simulink model "AFC_FFNN_trainscg_15_15_15_15_15_ctr_Nor_July_15"  (R2021a)
settings: Solver=VariableStepAuto  StartTime=0.0  StopTime=10.0  RelTol=1e-3
libraries: neural x82
(part 1 of 3)
settings Model: Creator=deyun  LastModifiedBy=deyun

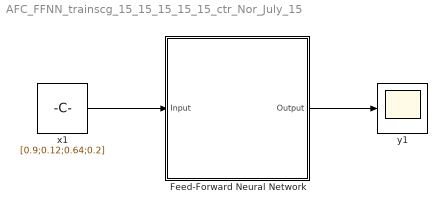
== system AFC_FFNN_trainscg_15_15_15_15_15_ctr_Nor_July_15 ==
  Feed-Forward Neural Network : Subsystem
      mask help: Feed-Forward Neural Network
      mask Display: e = 0.06;c1 = [120 150 230]/255;c2 = ([120 150 230]+0)/383;c3 = ([120 150 230]+128)/383;patch([0 1 1 0],[0 0 1 1],c1);patch([0 1 1 1-e 1-e 0+e],[0 0 1 1-e 0+e 0+e],c2);patch([0 0 1 1-e 0+e 0+e],[0 1 1 1-e 1-e 0+e],c3);plot([0 1 1 0 0],[0 0 1 1 0]);fprintf('NNET');port_label('input',1,' Input');port_label('output',1,'Output ');
  x1 : Constant  Value=[0.9;0.12;0.64;0.2]  SampleTime=1
      mask Display: e = 0.06;c1 = [120 230 180]/255;c2 = ([120 230 180]+0)/(256+128);c3 = ([120 230 180]+128)/(256+128);patch([0 1 1 0],[0 0 1 1],c1);patch([0 1 1 1-e 1-e 0+e],[0 0 1 1-e 0+e 0+e],c2);patch([0 0 1 1-e 0+e 0+e],[0 1 1 1-e 1-e 0+e],c3);plot([0 1 1 0 0],[0 0 1 1 0]);disp('Constant');
  y1 : Scope
      mask Display: e = 0.06;c1 = [120 230 180]/255;c2 = ([120 230 180]+0)/(256+128);c3 = ([120 230 180]+128)/(256+128);patch([0 1 1 0],[0 0 1 1],c1);patch([0 1 1 1-e 1-e 0+e],[0 0 1 1-e 0+e 0+e],c2);patch([0 0 1 1-e 0+e 0+e],[0 1 1 1-e 1-e 0+e],c3);plot([0 1 1 0 0],[0 0 1 1 0]);plot([0.15 0.85 0.85 0.15 0.15],[0.5 0.5 0.85 0.85 0.5]);
  wires:
  x1/1 -> Feed-Forward Neural Network/1(Input)
  Feed-Forward Neural Network/1(Output) -> y1/1

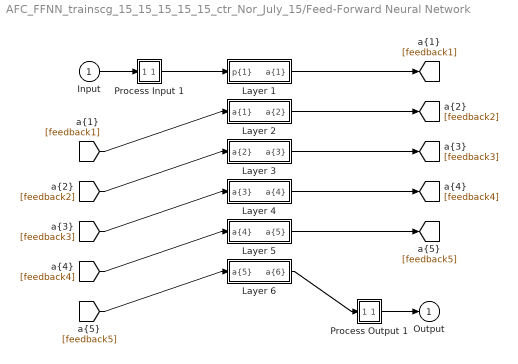
== system AFC_FFNN_trainscg_15_15_15_15_15_ctr_Nor_July_15/Feed-Forward Neural Network ==
  Input : Inport  PortDimensions=4
      mask Display: e = 0.06;c1 = [120 230 180]/255;c2 = ([120 230 180]+0)/(256+128);c3 = ([120 230 180]+128)/(256+128);patch([0 1 1 0],[0 0 1 1],c1);patch([0 1 1 1-e 1-e 0+e],[0 0 1 1-e 0+e 0+e],c2);patch([0 0 1 1-e 0+e 0+e],[0 1 1 1-e 1-e 0+e],c3);plot([0 1 1 0 0],[0 0 1 1 0]);
  Layer 1 : Subsystem
      mask Display: e = 0.06;c1 = [120 150 230]/255;c2 = ([120 150 230]+0)/383;c3 = ([120 150 230]+128)/383;patch([0 1 1 0],[0 0 1 1],c1);patch([0 1 1 1-e 1-e 0+e],[0 0 1 1-e 0+e 0+e],c2);patch([0 0 1 1-e 0+e 0+e],[0 1 1 1-e 1-e 0+e],c3);plot([0 1 1 0 0],[0 0 1 1 0]);
  Layer 2 : Subsystem
      mask Display: e = 0.06;c1 = [120 150 230]/255;c2 = ([120 150 230]+0)/383;c3 = ([120 150 230]+128)/383;patch([0 1 1 0],[0 0 1 1],c1);patch([0 1 1 1-e 1-e 0+e],[0 0 1 1-e 0+e 0+e],c2);patch([0 0 1 1-e 0+e 0+e],[0 1 1 1-e 1-e 0+e],c3);plot([0 1 1 0 0],[0 0 1 1 0]);
  Layer 3 : Subsystem
      mask Display: e = 0.06;c1 = [120 150 230]/255;c2 = ([120 150 230]+0)/383;c3 = ([120 150 230]+128)/383;patch([0 1 1 0],[0 0 1 1],c1);patch([0 1 1 1-e 1-e 0+e],[0 0 1 1-e 0+e 0+e],c2);patch([0 0 1 1-e 0+e 0+e],[0 1 1 1-e 1-e 0+e],c3);plot([0 1 1 0 0],[0 0 1 1 0]);
  Layer 4 : Subsystem
      mask Display: e = 0.06;c1 = [120 150 230]/255;c2 = ([120 150 230]+0)/383;c3 = ([120 150 230]+128)/383;patch([0 1 1 0],[0 0 1 1],c1);patch([0 1 1 1-e 1-e 0+e],[0 0 1 1-e 0+e 0+e],c2);patch([0 0 1 1-e 0+e 0+e],[0 1 1 1-e 1-e 0+e],c3);plot([0 1 1 0 0],[0 0 1 1 0]);
  Layer 5 : Subsystem
      mask Display: e = 0.06;c1 = [120 150 230]/255;c2 = ([120 150 230]+0)/383;c3 = ([120 150 230]+128)/383;patch([0 1 1 0],[0 0 1 1],c1);patch([0 1 1 1-e 1-e 0+e],[0 0 1 1-e 0+e 0+e],c2);patch([0 0 1 1-e 0+e 0+e],[0 1 1 1-e 1-e 0+e],c3);plot([0 1 1 0 0],[0 0 1 1 0]);
  Layer 6 : Subsystem
      mask Display: e = 0.06;c1 = [120 150 230]/255;c2 = ([120 150 230]+0)/383;c3 = ([120 150 230]+128)/383;patch([0 1 1 0],[0 0 1 1],c1);patch([0 1 1 1-e 1-e 0+e],[0 0 1 1-e 0+e 0+e],c2);patch([0 0 1 1-e 0+e 0+e],[0 1 1 1-e 1-e 0+e],c3);plot([0 1 1 0 0],[0 0 1 1 0]);
  Process Input 1 : Subsystem
      mask Display: e = 0.06;c1 = [120 150 230]/255;c2 = ([120 150 230]+0)/383;c3 = ([120 150 230]+128)/383;patch([0 1 1 0],[0 0 1 1],c1);patch([0 1 1 1-e 1-e 0+e],[0 0 1 1-e 0+e 0+e],c2);patch([0 0 1 1-e 0+e 0+e],[0 1 1 1-e 1-e 0+e],c3);plot([0 1 1 0 0],[0 0 1 1 0]);
  Process Output 1 : Subsystem
      mask Display: e = 0.06;c1 = [120 150 230]/255;c2 = ([120 150 230]+0)/383;c3 = ([120 150 230]+128)/383;patch([0 1 1 0],[0 0 1 1],c1);patch([0 1 1 1-e 1-e 0+e],[0 0 1 1-e 0+e 0+e],c2);patch([0 0 1 1-e 0+e 0+e],[0 1 1 1-e 1-e 0+e],c3);plot([0 1 1 0 0],[0 0 1 1 0]);
  Output : Outport  InitialOutput=0
      mask Display: e = 0.06;c1 = [120 230 180]/255;c2 = ([120 230 180]+0)/(256+128);c3 = ([120 230 180]+128)/(256+128);patch([0 1 1 0],[0 0 1 1],c1);patch([0 1 1 1-e 1-e 0+e],[0 0 1 1-e 0+e 0+e],c2);patch([0 0 1 1-e 0+e 0+e],[0 1 1 1-e 1-e 0+e],c3);plot([0 1 1 0 0],[0 0 1 1 0]);
  wires:
  Input/1 -> Process Input 1/1(x)
  Process Output 1/1(y) -> Output/1
  Process Input 1/1(p) -> Layer 1/1("p{1}")
  Layer 1/1("a{1}") -> [feedback1]
  [feedback1] -> Layer 2/1("a{1} ")
  Layer 2/1("a{2}") -> [feedback2]
  [feedback2] -> Layer 3/1("a{2} ")
  Layer 3/1("a{3}") -> [feedback3]
  [feedback3] -> Layer 4/1("a{3} ")
  Layer 4/1("a{4}") -> [feedback4]
  [feedback4] -> Layer 5/1("a{4} ")
  Layer 5/1("a{5}") -> [feedback5]
  [feedback5] -> Layer 6/1("a{5} ")
  Layer 6/1("a{6}") -> Process Output 1/1(a)

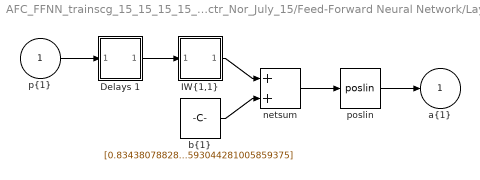
== system AFC_FFNN_trainscg_15_15_15_15_15_ctr_Nor_July_15/Feed-Forward Neural Network/Layer 1 ==
  "p{1}" : Inport  PortDimensions=4
      mask Display: e = 0.06;c1 = [120 230 180]/255;c2 = ([120 230 180]+0)/(256+128);c3 = ([120 230 180]+128)/(256+128);patch([0 1 1 0],[0 0 1 1],c1);patch([0 1 1 1-e 1-e 0+e],[0 0 1 1-e 0+e 0+e],c2);patch([0 0 1 1-e 0+e 0+e],[0 1 1 1-e 1-e 0+e],c3);plot([0 1 1 0 0],[0 0 1 1 0]);
  Delays 1 : Subsystem
      mask Display: e = 0.06;c1 = [120 150 230]/255;c2 = ([120 150 230]+0)/383;c3 = ([120 150 230]+128)/383;patch([0 1 1 0],[0 0 1 1],c1);patch([0 1 1 1-e 1-e 0+e],[0 0 1 1-e 0+e 0+e],c2);patch([0 0 1 1-e 0+e 0+e],[0 1 1 1-e 1-e 0+e],c3);plot([0 1 1 0 0],[0 0 1 1 0]);disp('0');
  "IW{1,1}" : Subsystem
      mask Display: e = 0.06;c1 = [120 150 230]/255;c2 = ([120 150 230]+0)/383;c3 = ([120 150 230]+128)/383;patch([0 1 1 0],[0 0 1 1],c1);patch([0 1 1 1-e 1-e 0+e],[0 0 1 1-e 0+e 0+e],c2);patch([0 0 1 1-e 0+e 0+e],[0 1 1 1-e 1-e 0+e],c3);plot([0 1 1 0 0],[0 0 1 1 0]);disp('W');
  "b{1}" : Constant  Value=[0.834380788285792096559134733979590237140655517578125;0.1683708190573824647895406769748660735785961151123046875;-0.5836974369680014707029158671502955257892608642578125;0.338402158427387023120758158256649039685726165771484375;0.3649283348189928943838822306133806705474853515625;-0.99006057888756249241168916341848671436309814453125;0.708204135272876289519672354799695312976837158203125;0.29241342293287486686637066668481566011905670166015625;-0.126123492443120099881781470685382373631000518798828125;0.049330225054286476471521183384538744576275348663330078125;0.376333591026828451209240711250458844006061553955078125;0.7508714290515745570786521057016216218471527099609375;-0.1970475991930808190577550931266159750521183013916015625;0.8830798190139279579824460597592405974864959716796875;0.50809102010338091925945036564371548593044281005859375]
      mask Display: e = 0.06;c1 = [120 150 230]/255;c2 = ([120 150 230]+0)/383;c3 = ([120 150 230]+128)/383;patch([0 1 1 0],[0 0 1 1],c1);patch([0 1 1 1-e 1-e 0+e],[0 0 1 1-e 0+e 0+e],c2);patch([0 0 1 1-e 0+e 0+e],[0 1 1 1-e 1-e 0+e],c3);plot([0 1 1 0 0],[0 0 1 1 0]);disp('b');
  netsum : Sum  Inputs=2  InputSameDT=on  SaturateOnIntegerOverflow=on  OutDataTypeStr=Inherit: Same as first input
      mask Display: e = 0.06;c1 = [120 150 230]/255;c2 = ([120 150 230]+0)/383;c3 = ([120 150 230]+128)/383;patch([0 1 1 0],[0 0 1 1],c1);patch([0 1 1 1-e 1-e 0+e],[0 0 1 1-e 0+e 0+e],c2);patch([0 0 1 1-e 0+e 0+e],[0 1 1 1-e 1-e 0+e],c3);plot([0 1 1 0 0],[0 0 1 1 0]);disp('+');
  poslin : neural/Transfer Functions/poslin
      settings: SourceProductBaseCode=NN
  "a{1}" : Outport  InitialOutput=[0;0;0;0;0;0;0;0;0;0;0;0;0;0;0]
      mask Display: e = 0.06;c1 = [120 230 180]/255;c2 = ([120 230 180]+0)/(256+128);c3 = ([120 230 180]+128)/(256+128);patch([0 1 1 0],[0 0 1 1],c1);patch([0 1 1 1-e 1-e 0+e],[0 0 1 1-e 0+e 0+e],c2);patch([0 0 1 1-e 0+e 0+e],[0 1 1 1-e 1-e 0+e],c3);plot([0 1 1 0 0],[0 0 1 1 0]);
  wires:
  "p{1}"/1 -> Delays 1/1("p{1}")
  Delays 1/1("pd{1,1}") -> "IW{1,1}"/1("pd{1,1}")
  "IW{1,1}"/1("iz{1,1}") -> netsum/1
  "b{1}"/1 -> netsum/2
  netsum/1 -> poslin/1
  poslin/1 -> "a{1}"/1

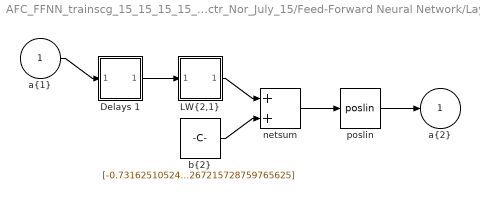
== system AFC_FFNN_trainscg_15_15_15_15_15_ctr_Nor_July_15/Feed-Forward Neural Network/Layer 2 ==
  "a{1} " : Inport  PortDimensions=15
      mask Display: e = 0.06;c1 = [120 230 180]/255;c2 = ([120 230 180]+0)/(256+128);c3 = ([120 230 180]+128)/(256+128);patch([0 1 1 0],[0 0 1 1],c1);patch([0 1 1 1-e 1-e 0+e],[0 0 1 1-e 0+e 0+e],c2);patch([0 0 1 1-e 0+e 0+e],[0 1 1 1-e 1-e 0+e],c3);plot([0 1 1 0 0],[0 0 1 1 0]);
  Delays 1 : Subsystem
      mask Display: e = 0.06;c1 = [120 150 230]/255;c2 = ([120 150 230]+0)/383;c3 = ([120 150 230]+128)/383;patch([0 1 1 0],[0 0 1 1],c1);patch([0 1 1 1-e 1-e 0+e],[0 0 1 1-e 0+e 0+e],c2);patch([0 0 1 1-e 0+e 0+e],[0 1 1 1-e 1-e 0+e],c3);plot([0 1 1 0 0],[0 0 1 1 0]);disp('0');
  "LW{2,1}" : Subsystem
      mask Display: e = 0.06;c1 = [120 150 230]/255;c2 = ([120 150 230]+0)/383;c3 = ([120 150 230]+128)/383;patch([0 1 1 0],[0 0 1 1],c1);patch([0 1 1 1-e 1-e 0+e],[0 0 1 1-e 0+e 0+e],c2);patch([0 0 1 1-e 0+e 0+e],[0 1 1 1-e 1-e 0+e],c3);plot([0 1 1 0 0],[0 0 1 1 0]);disp('W');
  "b{2}" : Constant  Value=[-0.731625105243399076471177977509796619415283203125;0.98363549254969495638789567237836308777332305908203125;-0.4406921090552768927040006019524298608303070068359375;-0.0487777105677955347129426399988005869090557098388671875;-0.9781485631689317283843365657958202064037322998046875;-0.2181690651886477871901348635219619609415531158447265625;0.650752066391559136349087566486559808254241943359375;-0.629923370383241643111205121385864913463592529296875;-0.1304003448000290443786752803134731948375701904296875;0.70007376089885064995854691005661152303218841552734375;-0.2715828071677421906571225918014533817768096923828125;-0.73112606194136187109933189276489429175853729248046875;-0.6072319242695296548362193789216689765453338623046875;0.62922478565097506031378316038171760737895965576171875;0.3126612773905483866343502086238004267215728759765625]
      mask Display: e = 0.06;c1 = [120 150 230]/255;c2 = ([120 150 230]+0)/383;c3 = ([120 150 230]+128)/383;patch([0 1 1 0],[0 0 1 1],c1);patch([0 1 1 1-e 1-e 0+e],[0 0 1 1-e 0+e 0+e],c2);patch([0 0 1 1-e 0+e 0+e],[0 1 1 1-e 1-e 0+e],c3);plot([0 1 1 0 0],[0 0 1 1 0]);disp('b');
  netsum : Sum  Inputs=2  InputSameDT=on  SaturateOnIntegerOverflow=on  OutDataTypeStr=Inherit: Same as first input
      mask Display: e = 0.06;c1 = [120 150 230]/255;c2 = ([120 150 230]+0)/383;c3 = ([120 150 230]+128)/383;patch([0 1 1 0],[0 0 1 1],c1);patch([0 1 1 1-e 1-e 0+e],[0 0 1 1-e 0+e 0+e],c2);patch([0 0 1 1-e 0+e 0+e],[0 1 1 1-e 1-e 0+e],c3);plot([0 1 1 0 0],[0 0 1 1 0]);disp('+');
  poslin : neural/Transfer Functions/poslin
      settings: SourceProductBaseCode=NN
  "a{2}" : Outport  InitialOutput=[0;0;0;0;0;0;0;0;0;0;0;0;0;0;0]
      mask Display: e = 0.06;c1 = [120 230 180]/255;c2 = ([120 230 180]+0)/(256+128);c3 = ([120 230 180]+128)/(256+128);patch([0 1 1 0],[0 0 1 1],c1);patch([0 1 1 1-e 1-e 0+e],[0 0 1 1-e 0+e 0+e],c2);patch([0 0 1 1-e 0+e 0+e],[0 1 1 1-e 1-e 0+e],c3);plot([0 1 1 0 0],[0 0 1 1 0]);
  wires:
  "a{1} "/1 -> Delays 1/1("p{2}")
  Delays 1/1("pd{2,1}") -> "LW{2,1}"/1("ad{2,1}")
  "LW{2,1}"/1("lz{2,1}") -> netsum/1
  "b{2}"/1 -> netsum/2
  netsum/1 -> poslin/1
  poslin/1 -> "a{2}"/1

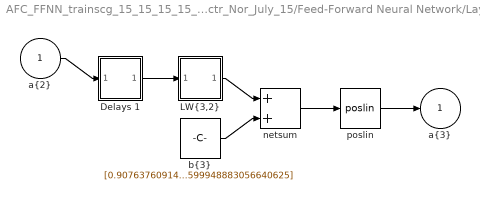
== system AFC_FFNN_trainscg_15_15_15_15_15_ctr_Nor_July_15/Feed-Forward Neural Network/Layer 3 ==
  "a{2} " : Inport  PortDimensions=15
      mask Display: e = 0.06;c1 = [120 230 180]/255;c2 = ([120 230 180]+0)/(256+128);c3 = ([120 230 180]+128)/(256+128);patch([0 1 1 0],[0 0 1 1],c1);patch([0 1 1 1-e 1-e 0+e],[0 0 1 1-e 0+e 0+e],c2);patch([0 0 1 1-e 0+e 0+e],[0 1 1 1-e 1-e 0+e],c3);plot([0 1 1 0 0],[0 0 1 1 0]);
  Delays 1 : Subsystem
      mask Display: e = 0.06;c1 = [120 150 230]/255;c2 = ([120 150 230]+0)/383;c3 = ([120 150 230]+128)/383;patch([0 1 1 0],[0 0 1 1],c1);patch([0 1 1 1-e 1-e 0+e],[0 0 1 1-e 0+e 0+e],c2);patch([0 0 1 1-e 0+e 0+e],[0 1 1 1-e 1-e 0+e],c3);plot([0 1 1 0 0],[0 0 1 1 0]);disp('0');
  "LW{3,2}" : Subsystem
      mask Display: e = 0.06;c1 = [120 150 230]/255;c2 = ([120 150 230]+0)/383;c3 = ([120 150 230]+128)/383;patch([0 1 1 0],[0 0 1 1],c1);patch([0 1 1 1-e 1-e 0+e],[0 0 1 1-e 0+e 0+e],c2);patch([0 0 1 1-e 0+e 0+e],[0 1 1 1-e 1-e 0+e],c3);plot([0 1 1 0 0],[0 0 1 1 0]);disp('W');
  "b{3}" : Constant  Value=[0.9076376091448159488805913497344590723514556884765625;-0.71600968460318714647883098223246634006500244140625;-0.471791323827774833343795535256504081189632415771484375;0.8981803810516881814152156948694027960300445556640625;0.57279257682278783558871282366453669965267181396484375;-0.0503326060717912415753971799858845770359039306640625;-0.15910530258065891384688939069746993482112884521484375;-0.3270770698152742905762124792090617120265960693359375;-0.9940373878755133230100682339980266988277435302734375;-0.0863911705552550535092137806714163161814212799072265625;0.460191396222384752068279567538411356508731842041015625;-0.9685414138824135488192723641986958682537078857421875;0.61396774169837142753891612301231361925601959228515625;-0.8178168206000091533525164777529425919055938720703125;-0.95450255486567758822502582916058599948883056640625]
      mask Display: e = 0.06;c1 = [120 150 230]/255;c2 = ([120 150 230]+0)/383;c3 = ([120 150 230]+128)/383;patch([0 1 1 0],[0 0 1 1],c1);patch([0 1 1 1-e 1-e 0+e],[0 0 1 1-e 0+e 0+e],c2);patch([0 0 1 1-e 0+e 0+e],[0 1 1 1-e 1-e 0+e],c3);plot([0 1 1 0 0],[0 0 1 1 0]);disp('b');
  netsum : Sum  Inputs=2  InputSameDT=on  SaturateOnIntegerOverflow=on  OutDataTypeStr=Inherit: Same as first input
      mask Display: e = 0.06;c1 = [120 150 230]/255;c2 = ([120 150 230]+0)/383;c3 = ([120 150 230]+128)/383;patch([0 1 1 0],[0 0 1 1],c1);patch([0 1 1 1-e 1-e 0+e],[0 0 1 1-e 0+e 0+e],c2);patch([0 0 1 1-e 0+e 0+e],[0 1 1 1-e 1-e 0+e],c3);plot([0 1 1 0 0],[0 0 1 1 0]);disp('+');
  poslin : neural/Transfer Functions/poslin
      settings: SourceProductBaseCode=NN
  "a{3}" : Outport  InitialOutput=[0;0;0;0;0;0;0;0;0;0;0;0;0;0;0]
      mask Display: e = 0.06;c1 = [120 230 180]/255;c2 = ([120 230 180]+0)/(256+128);c3 = ([120 230 180]+128)/(256+128);patch([0 1 1 0],[0 0 1 1],c1);patch([0 1 1 1-e 1-e 0+e],[0 0 1 1-e 0+e 0+e],c2);patch([0 0 1 1-e 0+e 0+e],[0 1 1 1-e 1-e 0+e],c3);plot([0 1 1 0 0],[0 0 1 1 0]);
  wires:
  "a{2} "/1 -> Delays 1/1("p{3}")
  Delays 1/1("pd{3,2}") -> "LW{3,2}"/1("ad{3,2}")
  "LW{3,2}"/1("lz{3,2}") -> netsum/1
  "b{3}"/1 -> netsum/2
  netsum/1 -> poslin/1
  poslin/1 -> "a{3}"/1

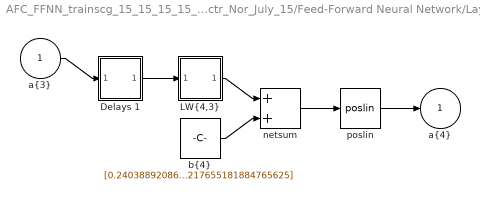
== system AFC_FFNN_trainscg_15_15_15_15_15_ctr_Nor_July_15/Feed-Forward Neural Network/Layer 4 ==
  "a{3} " : Inport  PortDimensions=15
      mask Display: e = 0.06;c1 = [120 230 180]/255;c2 = ([120 230 180]+0)/(256+128);c3 = ([120 230 180]+128)/(256+128);patch([0 1 1 0],[0 0 1 1],c1);patch([0 1 1 1-e 1-e 0+e],[0 0 1 1-e 0+e 0+e],c2);patch([0 0 1 1-e 0+e 0+e],[0 1 1 1-e 1-e 0+e],c3);plot([0 1 1 0 0],[0 0 1 1 0]);
  Delays 1 : Subsystem
      mask Display: e = 0.06;c1 = [120 150 230]/255;c2 = ([120 150 230]+0)/383;c3 = ([120 150 230]+128)/383;patch([0 1 1 0],[0 0 1 1],c1);patch([0 1 1 1-e 1-e 0+e],[0 0 1 1-e 0+e 0+e],c2);patch([0 0 1 1-e 0+e 0+e],[0 1 1 1-e 1-e 0+e],c3);plot([0 1 1 0 0],[0 0 1 1 0]);disp('0');
  "LW{4,3}" : Subsystem
      mask Display: e = 0.06;c1 = [120 150 230]/255;c2 = ([120 150 230]+0)/383;c3 = ([120 150 230]+128)/383;patch([0 1 1 0],[0 0 1 1],c1);patch([0 1 1 1-e 1-e 0+e],[0 0 1 1-e 0+e 0+e],c2);patch([0 0 1 1-e 0+e 0+e],[0 1 1 1-e 1-e 0+e],c3);plot([0 1 1 0 0],[0 0 1 1 0]);disp('W');
  "b{4}" : Constant  Value=[0.240388920861316635058102519906242378056049346923828125;-0.54165698217604385522605525693506933748722076416015625;-0.88616717557675583893939119661808945238590240478515625;0.7745823050006988008675534729263745248317718505859375;-0.45280715027888351897900065523572266101837158203125;-0.2071610134627379640193112209090031683444976806640625;-0.54495312574752297063440664715017192065715789794921875;0.880939944409394382063283046591095626354217529296875;-0.71516380216721608942265220321132801473140716552734375;-0.76460765353241288977415024419315159320831298828125;-0.4747463081831833076051907482906244695186614990234375;-0.381511549098789093381611792210605926811695098876953125;-0.66200180902120087100826140158460475504398345947265625;0.40957019446229814274573755028541199862957000732421875;0.69878230535015595226155937780276872217655181884765625]
      mask Display: e = 0.06;c1 = [120 150 230]/255;c2 = ([120 150 230]+0)/383;c3 = ([120 150 230]+128)/383;patch([0 1 1 0],[0 0 1 1],c1);patch([0 1 1 1-e 1-e 0+e],[0 0 1 1-e 0+e 0+e],c2);patch([0 0 1 1-e 0+e 0+e],[0 1 1 1-e 1-e 0+e],c3);plot([0 1 1 0 0],[0 0 1 1 0]);disp('b');
  netsum : Sum  Inputs=2  InputSameDT=on  SaturateOnIntegerOverflow=on  OutDataTypeStr=Inherit: Same as first input
      mask Display: e = 0.06;c1 = [120 150 230]/255;c2 = ([120 150 230]+0)/383;c3 = ([120 150 230]+128)/383;patch([0 1 1 0],[0 0 1 1],c1);patch([0 1 1 1-e 1-e 0+e],[0 0 1 1-e 0+e 0+e],c2);patch([0 0 1 1-e 0+e 0+e],[0 1 1 1-e 1-e 0+e],c3);plot([0 1 1 0 0],[0 0 1 1 0]);disp('+');
  poslin : neural/Transfer Functions/poslin
      settings: SourceProductBaseCode=NN
  "a{4}" : Outport  InitialOutput=[0;0;0;0;0;0;0;0;0;0;0;0;0;0;0]
      mask Display: e = 0.06;c1 = [120 230 180]/255;c2 = ([120 230 180]+0)/(256+128);c3 = ([120 230 180]+128)/(256+128);patch([0 1 1 0],[0 0 1 1],c1);patch([0 1 1 1-e 1-e 0+e],[0 0 1 1-e 0+e 0+e],c2);patch([0 0 1 1-e 0+e 0+e],[0 1 1 1-e 1-e 0+e],c3);plot([0 1 1 0 0],[0 0 1 1 0]);
  wires:
  "a{3} "/1 -> Delays 1/1("p{4}")
  Delays 1/1("pd{4,3}") -> "LW{4,3}"/1("ad{4,3}")
  "LW{4,3}"/1("lz{4,3}") -> netsum/1
  "b{4}"/1 -> netsum/2
  netsum/1 -> poslin/1
  poslin/1 -> "a{4}"/1

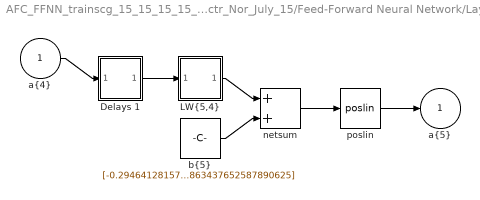
== system AFC_FFNN_trainscg_15_15_15_15_15_ctr_Nor_July_15/Feed-Forward Neural Network/Layer 5 ==
  "a{4} " : Inport  PortDimensions=15
      mask Display: e = 0.06;c1 = [120 230 180]/255;c2 = ([120 230 180]+0)/(256+128);c3 = ([120 230 180]+128)/(256+128);patch([0 1 1 0],[0 0 1 1],c1);patch([0 1 1 1-e 1-e 0+e],[0 0 1 1-e 0+e 0+e],c2);patch([0 0 1 1-e 0+e 0+e],[0 1 1 1-e 1-e 0+e],c3);plot([0 1 1 0 0],[0 0 1 1 0]);
  Delays 1 : Subsystem
      mask Display: e = 0.06;c1 = [120 150 230]/255;c2 = ([120 150 230]+0)/383;c3 = ([120 150 230]+128)/383;patch([0 1 1 0],[0 0 1 1],c1);patch([0 1 1 1-e 1-e 0+e],[0 0 1 1-e 0+e 0+e],c2);patch([0 0 1 1-e 0+e 0+e],[0 1 1 1-e 1-e 0+e],c3);plot([0 1 1 0 0],[0 0 1 1 0]);disp('0');
  "LW{5,4}" : Subsystem
      mask Display: e = 0.06;c1 = [120 150 230]/255;c2 = ([120 150 230]+0)/383;c3 = ([120 150 230]+128)/383;patch([0 1 1 0],[0 0 1 1],c1);patch([0 1 1 1-e 1-e 0+e],[0 0 1 1-e 0+e 0+e],c2);patch([0 0 1 1-e 0+e 0+e],[0 1 1 1-e 1-e 0+e],c3);plot([0 1 1 0 0],[0 0 1 1 0]);disp('W');
  "b{5}" : Constant  Value=[-0.2946412815799941409267148628714494407176971435546875;0.1595872947699004396060473709439975209534168243408203125;0.8822615072154018633909799973480403423309326171875;0.475423242355577979623149076360277831554412841796875;0.421121879353651251687296053205500356853008270263671875;0.6612140130957249173349055126891471445560455322265625;0.6756659893504315395063031246536411345005035400390625;-0.2966656234565057115304398394073359668254852294921875;0.732279491352301192819140851497650146484375;0.040781724623681910035788433788184192962944507598876953125;0.2887224456675550054995937898638658225536346435546875;-0.4415456635376120431146773626096546649932861328125;-0.1640940243245461171994747928692959249019622802734375;-0.50284217825491561715267607723944820463657379150390625;0.525205747767737651798825027071870863437652587890625]
      mask Display: e = 0.06;c1 = [120 150 230]/255;c2 = ([120 150 230]+0)/383;c3 = ([120 150 230]+128)/383;patch([0 1 1 0],[0 0 1 1],c1);patch([0 1 1 1-e 1-e 0+e],[0 0 1 1-e 0+e 0+e],c2);patch([0 0 1 1-e 0+e 0+e],[0 1 1 1-e 1-e 0+e],c3);plot([0 1 1 0 0],[0 0 1 1 0]);disp('b');
  netsum : Sum  Inputs=2  InputSameDT=on  SaturateOnIntegerOverflow=on  OutDataTypeStr=Inherit: Same as first input
      mask Display: e = 0.06;c1 = [120 150 230]/255;c2 = ([120 150 230]+0)/383;c3 = ([120 150 230]+128)/383;patch([0 1 1 0],[0 0 1 1],c1);patch([0 1 1 1-e 1-e 0+e],[0 0 1 1-e 0+e 0+e],c2);patch([0 0 1 1-e 0+e 0+e],[0 1 1 1-e 1-e 0+e],c3);plot([0 1 1 0 0],[0 0 1 1 0]);disp('+');
  poslin : neural/Transfer Functions/poslin
      settings: SourceProductBaseCode=NN
  "a{5}" : Outport  InitialOutput=[0;0;0;0;0;0;0;0;0;0;0;0;0;0;0]
      mask Display: e = 0.06;c1 = [120 230 180]/255;c2 = ([120 230 180]+0)/(256+128);c3 = ([120 230 180]+128)/(256+128);patch([0 1 1 0],[0 0 1 1],c1);patch([0 1 1 1-e 1-e 0+e],[0 0 1 1-e 0+e 0+e],c2);patch([0 0 1 1-e 0+e 0+e],[0 1 1 1-e 1-e 0+e],c3);plot([0 1 1 0 0],[0 0 1 1 0]);
  wires:
  "a{4} "/1 -> Delays 1/1("p{5}")
  Delays 1/1("pd{5,4}") -> "LW{5,4}"/1("ad{5,4}")
  "LW{5,4}"/1("lz{5,4}") -> netsum/1
  "b{5}"/1 -> netsum/2
  netsum/1 -> poslin/1
  poslin/1 -> "a{5}"/1

== system AFC_FFNN_trainscg_15_15_15_15_15_ctr_Nor_July_15/Feed-Forward Neural Network/Layer 6 ==
  "a{5} " : Inport  PortDimensions=15
      mask Display: e = 0.06;c1 = [120 230 180]/255;c2 = ([120 230 180]+0)/(256+128);c3 = ([120 230 180]+128)/(256+128);patch([0 1 1 0],[0 0 1 1],c1);patch([0 1 1 1-e 1-e 0+e],[0 0 1 1-e 0+e 0+e],c2);patch([0 0 1 1-e 0+e 0+e],[0 1 1 1-e 1-e 0+e],c3);plot([0 1 1 0 0],[0 0 1 1 0]);
  Delays 1 : Subsystem
      mask Display: e = 0.06;c1 = [120 150 230]/255;c2 = ([120 150 230]+0)/383;c3 = ([120 150 230]+128)/383;patch([0 1 1 0],[0 0 1 1],c1);patch([0 1 1 1-e 1-e 0+e],[0 0 1 1-e 0+e 0+e],c2);patch([0 0 1 1-e 0+e 0+e],[0 1 1 1-e 1-e 0+e],c3);plot([0 1 1 0 0],[0 0 1 1 0]);disp('0');
  "LW{6,5}" : Subsystem
      mask Display: e = 0.06;c1 = [120 150 230]/255;c2 = ([120 150 230]+0)/383;c3 = ([120 150 230]+128)/383;patch([0 1 1 0],[0 0 1 1],c1);patch([0 1 1 1-e 1-e 0+e],[0 0 1 1-e 0+e 0+e],c2);patch([0 0 1 1-e 0+e 0+e],[0 1 1 1-e 1-e 0+e],c3);plot([0 1 1 0 0],[0 0 1 1 0]);disp('W');
  "b{6}" : Constant  Value=0.47753318153695001324621216554078273475170135498046875
      mask Display: e = 0.06;c1 = [120 150 230]/255;c2 = ([120 150 230]+0)/383;c3 = ([120 150 230]+128)/383;patch([0 1 1 0],[0 0 1 1],c1);patch([0 1 1 1-e 1-e 0+e],[0 0 1 1-e 0+e 0+e],c2);patch([0 0 1 1-e 0+e 0+e],[0 1 1 1-e 1-e 0+e],c3);plot([0 1 1 0 0],[0 0 1 1 0]);disp('b');
  netsum : Sum  Inputs=2  InputSameDT=on  SaturateOnIntegerOverflow=on  OutDataTypeStr=Inherit: Same as first input
      mask Display: e = 0.06;c1 = [120 150 230]/255;c2 = ([120 150 230]+0)/383;c3 = ([120 150 230]+128)/383;patch([0 1 1 0],[0 0 1 1],c1);patch([0 1 1 1-e 1-e 0+e],[0 0 1 1-e 0+e 0+e],c2);patch([0 0 1 1-e 0+e 0+e],[0 1 1 1-e 1-e 0+e],c3);plot([0 1 1 0 0],[0 0 1 1 0]);disp('+');
  purelin : neural/Transfer Functions/purelin
  "a{6}" : Outport  InitialOutput=0
      mask Display: e = 0.06;c1 = [120 230 180]/255;c2 = ([120 230 180]+0)/(256+128);c3 = ([120 230 180]+128)/(256+128);patch([0 1 1 0],[0 0 1 1],c1);patch([0 1 1 1-e 1-e 0+e],[0 0 1 1-e 0+e 0+e],c2);patch([0 0 1 1-e 0+e 0+e],[0 1 1 1-e 1-e 0+e],c3);plot([0 1 1 0 0],[0 0 1 1 0]);
  wires:
  "a{5} "/1 -> Delays 1/1("p{6}")
  Delays 1/1("pd{6,5}") -> "LW{6,5}"/1("ad{6,5}")
  "LW{6,5}"/1("lz{6,5}") -> netsum/1
  "b{6}"/1 -> netsum/2
  netsum/1 -> purelin/1
  purelin/1 -> "a{6}"/1

== system AFC_FFNN_trainscg_15_15_15_15_15_ctr_Nor_July_15/Feed-Forward Neural Network/Process Input 1 ==
  x : Inport  PortDimensions=4
      mask Display: e = 0.06;c1 = [120 230 180]/255;c2 = ([120 230 180]+0)/(256+128);c3 = ([120 230 180]+128)/(256+128);patch([0 1 1 0],[0 0 1 1],c1);patch([0 1 1 1-e 1-e 0+e],[0 0 1 1-e 0+e 0+e],c2);patch([0 0 1 1-e 0+e 0+e],[0 1 1 1-e 1-e 0+e],c3);plot([0 1 1 0 0],[0 0 1 1 0]);
  p : Outport  PortDimensions=4
      mask Display: e = 0.06;c1 = [120 230 180]/255;c2 = ([120 230 180]+0)/(256+128);c3 = ([120 230 180]+128)/(256+128);patch([0 1 1 0],[0 0 1 1],c1);patch([0 1 1 1-e 1-e 0+e],[0 0 1 1-e 0+e 0+e],c2);patch([0 0 1 1-e 0+e 0+e],[0 1 1 1-e 1-e 0+e],c3);plot([0 1 1 0 0],[0 0 1 1 0]);
  wires:
  x/1 -> p/1

== system AFC_FFNN_trainscg_15_15_15_15_15_ctr_Nor_July_15/Feed-Forward Neural Network/Process Output 1 ==
  a : Inport  PortDimensions=1
      mask Display: e = 0.06;c1 = [120 230 180]/255;c2 = ([120 230 180]+0)/(256+128);c3 = ([120 230 180]+128)/(256+128);patch([0 1 1 0],[0 0 1 1],c1);patch([0 1 1 1-e 1-e 0+e],[0 0 1 1-e 0+e 0+e],c2);patch([0 0 1 1-e 0+e 0+e],[0 1 1 1-e 1-e 0+e],c3);plot([0 1 1 0 0],[0 0 1 1 0]);
  y : Outport  PortDimensions=1
      mask Display: e = 0.06;c1 = [120 230 180]/255;c2 = ([120 230 180]+0)/(256+128);c3 = ([120 230 180]+128)/(256+128);patch([0 1 1 0],[0 0 1 1],c1);patch([0 1 1 1-e 1-e 0+e],[0 0 1 1-e 0+e 0+e],c2);patch([0 0 1 1-e 0+e 0+e],[0 1 1 1-e 1-e 0+e],c3);plot([0 1 1 0 0],[0 0 1 1 0]);
  wires:
  a/1 -> y/1

== system AFC_FFNN_trainscg_15_15_15_15_15_ctr_Nor_July_15/Feed-Forward Neural Network/Layer 1/Delays 1 ==
  "p{1}" : Inport  PortDimensions=4
      mask Display: e = 0.06;c1 = [120 230 180]/255;c2 = ([120 230 180]+0)/(256+128);c3 = ([120 230 180]+128)/(256+128);patch([0 1 1 0],[0 0 1 1],c1);patch([0 1 1 1-e 1-e 0+e],[0 0 1 1-e 0+e 0+e],c2);patch([0 0 1 1-e 0+e 0+e],[0 1 1 1-e 1-e 0+e],c3);plot([0 1 1 0 0],[0 0 1 1 0]);
  mux : Mux  Inputs=1
      mask Display: e = 0.06;c1 = [120 150 230]/255;c2 = ([120 150 230]+0)/383;c3 = ([120 150 230]+128)/383;patch([0 1 1 0],[0 0 1 1],c1);patch([0 1 1 1-e 1-e 0+e],[0 0 1 1-e 0+e 0+e],c2);patch([0 0 1 1-e 0+e 0+e],[0 1 1 1-e 1-e 0+e],c3);plot([0 1 1 0 0],[0 0 1 1 0]);disp('Mux')
  "pd{1,1}" : Outport
      mask Display: e = 0.06;c1 = [120 230 180]/255;c2 = ([120 230 180]+0)/(256+128);c3 = ([120 230 180]+128)/(256+128);patch([0 1 1 0],[0 0 1 1],c1);patch([0 1 1 1-e 1-e 0+e],[0 0 1 1-e 0+e 0+e],c2);patch([0 0 1 1-e 0+e 0+e],[0 1 1 1-e 1-e 0+e],c3);plot([0 1 1 0 0],[0 0 1 1 0]);
  wires:
  "p{1}"/1 -> mux/1
  mux/1 -> "pd{1,1}"/1

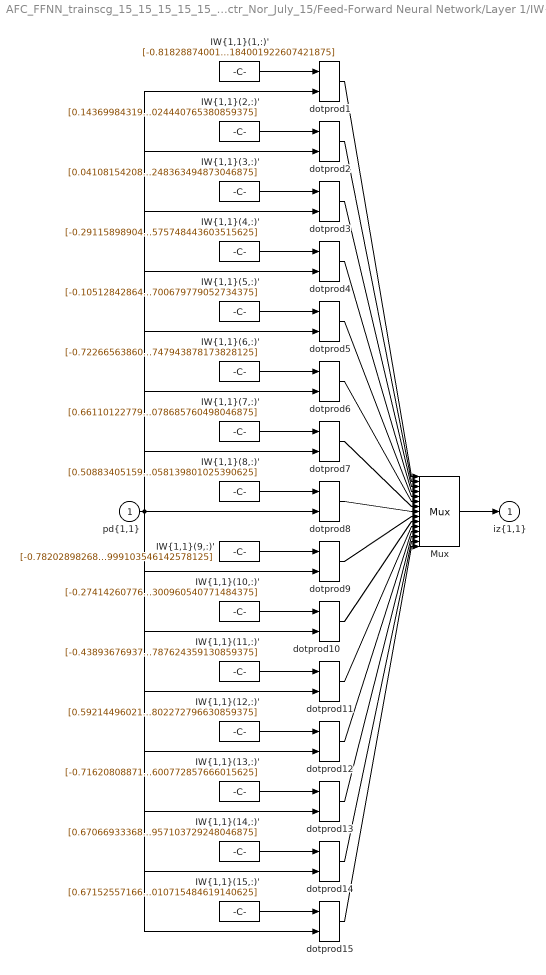
== system AFC_FFNN_trainscg_15_15_15_15_15_ctr_Nor_July_15/Feed-Forward Neural Network/Layer 1/IW{1,1} ==
  "pd{1,1}" : Inport  PortDimensions=4
      mask Display: e = 0.06;c1 = [120 230 180]/255;c2 = ([120 230 180]+0)/(256+128);c3 = ([120 230 180]+128)/(256+128);patch([0 1 1 0],[0 0 1 1],c1);patch([0 1 1 1-e 1-e 0+e],[0 0 1 1-e 0+e 0+e],c2);patch([0 0 1 1-e 0+e 0+e],[0 1 1 1-e 1-e 0+e],c3);plot([0 1 1 0 0],[0 0 1 1 0]);
  "IW{1,1}(1,:)'" : Constant  Value=[-0.8182887400167964120356600687955506145954132080078125;-0.49598144760943763120764060658984817564487457275390625;0.06041818616274809150556990289260284043848514556884765625;0.0133499737911447029226064131535167689435184001922607421875]
      mask Display: e = 0.06;c1 = [120 150 230]/255;c2 = ([120 150 230]+0)/383;c3 = ([120 150 230]+128)/383;patch([0 1 1 0],[0 0 1 1],c1);patch([0 1 1 1-e 1-e 0+e],[0 0 1 1-e 0+e 0+e],c2);patch([0 0 1 1-e 0+e 0+e],[0 1 1 1-e 1-e 0+e],c3);plot([0 1 1 0 0],[0 0 1 1 0]);disp('Weights');
  "IW{1,1}(10,:)'" : Constant  Value=[-0.274142607765400503350150529513484798371791839599609375;-0.353746335085151131227831911019166000187397003173828125;0.01179470110379924295551656854286193265579640865325927734375;0.099327920447423723171453957547782920300960540771484375]
      mask Display: e = 0.06;c1 = [120 150 230]/255;c2 = ([120 150 230]+0)/383;c3 = ([120 150 230]+128)/383;patch([0 1 1 0],[0 0 1 1],c1);patch([0 1 1 1-e 1-e 0+e],[0 0 1 1-e 0+e 0+e],c2);patch([0 0 1 1-e 0+e 0+e],[0 1 1 1-e 1-e 0+e],c3);plot([0 1 1 0 0],[0 0 1 1 0]);disp('Weights');
  "IW{1,1}(11,:)'" : Constant  Value=[-0.43893676937472270171980426312074996531009674072265625;0.1821822685096182448116763907819404266774654388427734375;0.69701670852280350754170967775280587375164031982421875;0.2445157951983446265042942968648276291787624359130859375]
      mask Display: e = 0.06;c1 = [120 150 230]/255;c2 = ([120 150 230]+0)/383;c3 = ([120 150 230]+128)/383;patch([0 1 1 0],[0 0 1 1],c1);patch([0 1 1 1-e 1-e 0+e],[0 0 1 1-e 0+e 0+e],c2);patch([0 0 1 1-e 0+e 0+e],[0 1 1 1-e 1-e 0+e],c3);plot([0 1 1 0 0],[0 0 1 1 0]);disp('Weights');
  "IW{1,1}(12,:)'" : Constant  Value=[0.59214496021067664077719427950796671211719512939453125;0.6211639297454680797017090299050323665142059326171875;0.45896429957388862330702750114141963422298431396484375;-0.71788574130490656610703581463894806802272796630859375]
      mask Display: e = 0.06;c1 = [120 150 230]/255;c2 = ([120 150 230]+0)/383;c3 = ([120 150 230]+128)/383;patch([0 1 1 0],[0 0 1 1],c1);patch([0 1 1 1-e 1-e 0+e],[0 0 1 1-e 0+e 0+e],c2);patch([0 0 1 1-e 0+e 0+e],[0 1 1 1-e 1-e 0+e],c3);plot([0 1 1 0 0],[0 0 1 1 0]);disp('Weights');
  "IW{1,1}(13,:)'" : Constant  Value=[-0.71620808871012420215862448458210565149784088134765625;0.4135587801428910470491473461152054369449615478515625;-0.289173209515923457235686555577558465301990509033203125;0.27039922822216144737694776267744600772857666015625]
      mask Display: e = 0.06;c1 = [120 150 230]/255;c2 = ([120 150 230]+0)/383;c3 = ([120 150 230]+128)/383;patch([0 1 1 0],[0 0 1 1],c1);patch([0 1 1 1-e 1-e 0+e],[0 0 1 1-e 0+e 0+e],c2);patch([0 0 1 1-e 0+e 0+e],[0 1 1 1-e 1-e 0+e],c3);plot([0 1 1 0 0],[0 0 1 1 0]);disp('Weights');
  "IW{1,1}(14,:)'" : Constant  Value=[0.67066933368885639499268336294335313141345977783203125;-0.453403126912178933149988324657897464931011199951171875;0.436183395002791851613466178605449385941028594970703125;0.4514754352094623168767384413513354957103729248046875]
      mask Display: e = 0.06;c1 = [120 150 230]/255;c2 = ([120 150 230]+0)/383;c3 = ([120 150 230]+128)/383;patch([0 1 1 0],[0 0 1 1],c1);patch([0 1 1 1-e 1-e 0+e],[0 0 1 1-e 0+e 0+e],c2);patch([0 0 1 1-e 0+e 0+e],[0 1 1 1-e 1-e 0+e],c3);plot([0 1 1 0 0],[0 0 1 1 0]);disp('Weights');
  "IW{1,1}(15,:)'" : Constant  Value=[0.6715255716655617046484394450089894235134124755859375;-0.887666042934819099485821425332687795162200927734375;-0.9589525699076890674632522859610617160797119140625;0.6290601453291844169513069573440589010715484619140625]
      mask Display: e = 0.06;c1 = [120 150 230]/255;c2 = ([120 150 230]+0)/383;c3 = ([120 150 230]+128)/383;patch([0 1 1 0],[0 0 1 1],c1);patch([0 1 1 1-e 1-e 0+e],[0 0 1 1-e 0+e 0+e],c2);patch([0 0 1 1-e 0+e 0+e],[0 1 1 1-e 1-e 0+e],c3);plot([0 1 1 0 0],[0 0 1 1 0]);disp('Weights');
  "IW{1,1}(2,:)'" : Constant  Value=[0.143699843190639720003076718057855032384395599365234375;-0.5405720325094571787616359870298765599727630615234375;-0.1096442863057018046735180405448772944509983062744140625;0.473688297171214356406920842346153222024440765380859375]
      mask Display: e = 0.06;c1 = [120 150 230]/255;c2 = ([120 150 230]+0)/383;c3 = ([120 150 230]+128)/383;patch([0 1 1 0],[0 0 1 1],c1);patch([0 1 1 1-e 1-e 0+e],[0 0 1 1-e 0+e 0+e],c2);patch([0 0 1 1-e 0+e 0+e],[0 1 1 1-e 1-e 0+e],c3);plot([0 1 1 0 0],[0 0 1 1 0]);disp('Weights');
  "IW{1,1}(3,:)'" : Constant  Value=[0.041081542089265621342519807512871921062469482421875;0.4871879533887997215657605920569039881229400634765625;-0.67363537454960553674254697398282587528228759765625;-0.2916475681070547221196420650812797248363494873046875]
      mask Display: e = 0.06;c1 = [120 150 230]/255;c2 = ([120 150 230]+0)/383;c3 = ([120 150 230]+128)/383;patch([0 1 1 0],[0 0 1 1],c1);patch([0 1 1 1-e 1-e 0+e],[0 0 1 1-e 0+e 0+e],c2);patch([0 0 1 1-e 0+e 0+e],[0 1 1 1-e 1-e 0+e],c3);plot([0 1 1 0 0],[0 0 1 1 0]);disp('Weights');
  "IW{1,1}(4,:)'" : Constant  Value=[-0.291158989040041060736285771781695075333118438720703125;0.85523357857572823714775722692138515412807464599609375;-0.343301083616170232826192432185052894055843353271484375;-0.164412991500933414190654957565129734575748443603515625]
      mask Display: e = 0.06;c1 = [120 150 230]/255;c2 = ([120 150 230]+0)/383;c3 = ([120 150 230]+128)/383;patch([0 1 1 0],[0 0 1 1],c1);patch([0 1 1 1-e 1-e 0+e],[0 0 1 1-e 0+e 0+e],c2);patch([0 0 1 1-e 0+e 0+e],[0 1 1 1-e 1-e 0+e],c3);plot([0 1 1 0 0],[0 0 1 1 0]);disp('Weights');
  "IW{1,1}(5,:)'" : Constant  Value=[-0.105128428648296246006310639131697826087474822998046875;0.365061060573851070554241005083895288407802581787109375;0.8346276011325670651785912923514842987060546875;0.09515404071335274716059160482473089359700679779052734375]
      mask Display: e = 0.06;c1 = [120 150 230]/255;c2 = ([120 150 230]+0)/383;c3 = ([120 150 230]+128)/383;patch([0 1 1 0],[0 0 1 1],c1);patch([0 1 1 1-e 1-e 0+e],[0 0 1 1-e 0+e 0+e],c2);patch([0 0 1 1-e 0+e 0+e],[0 1 1 1-e 1-e 0+e],c3);plot([0 1 1 0 0],[0 0 1 1 0]);disp('Weights');
  "IW{1,1}(6,:)'" : Constant  Value=[-0.722665638608478655413591695833019912242889404296875;0.985695769868679239067432718002237379550933837890625;-0.430803036254950644234895662521012127399444580078125;-0.8468350786113305606050971618969924747943878173828125]
      mask Display: e = 0.06;c1 = [120 150 230]/255;c2 = ([120 150 230]+0)/383;c3 = ([120 150 230]+128)/383;patch([0 1 1 0],[0 0 1 1],c1);patch([0 1 1 1-e 1-e 0+e],[0 0 1 1-e 0+e 0+e],c2);patch([0 0 1 1-e 0+e 0+e],[0 1 1 1-e 1-e 0+e],c3);plot([0 1 1 0 0],[0 0 1 1 0]);disp('Weights');
  "IW{1,1}(7,:)'" : Constant  Value=[0.66110122779032021167466837141546420753002166748046875;0.82898282548024060378821786798653192818164825439453125;0.72451838656569245156191527712508104741573333740234375;0.74217279844588712744979375202092342078685760498046875]
      mask Display: e = 0.06;c1 = [120 150 230]/255;c2 = ([120 150 230]+0)/383;c3 = ([120 150 230]+128)/383;patch([0 1 1 0],[0 0 1 1],c1);patch([0 1 1 1-e 1-e 0+e],[0 0 1 1-e 0+e 0+e],c2);patch([0 0 1 1-e 0+e 0+e],[0 1 1 1-e 1-e 0+e],c3);plot([0 1 1 0 0],[0 0 1 1 0]);disp('Weights');
  "IW{1,1}(8,:)'" : Constant  Value=[0.50883405159613970258902782006771303713321685791015625;0.594873705997945645407298798090778291225433349609375;-0.4681697843469925235382333994493819773197174072265625;0.492204681578230884841929082540445961058139801025390625]
      mask Display: e = 0.06;c1 = [120 150 230]/255;c2 = ([120 150 230]+0)/383;c3 = ([120 150 230]+128)/383;patch([0 1 1 0],[0 0 1 1],c1);patch([0 1 1 1-e 1-e 0+e],[0 0 1 1-e 0+e 0+e],c2);patch([0 0 1 1-e 0+e 0+e],[0 1 1 1-e 1-e 0+e],c3);plot([0 1 1 0 0],[0 0 1 1 0]);disp('Weights');
  "IW{1,1}(9,:)'" : Constant  Value=[-0.78202898268480403043412252372945658862590789794921875;0.85507523981980348981579709288780577480792999267578125;0.270272157299210558090152289878460578620433807373046875;-0.57478282284230808318881145169143564999103546142578125]
      mask Display: e = 0.06;c1 = [120 150 230]/255;c2 = ([120 150 230]+0)/383;c3 = ([120 150 230]+128)/383;patch([0 1 1 0],[0 0 1 1],c1);patch([0 1 1 1-e 1-e 0+e],[0 0 1 1-e 0+e 0+e],c2);patch([0 0 1 1-e 0+e 0+e],[0 1 1 1-e 1-e 0+e],c3);plot([0 1 1 0 0],[0 0 1 1 0]);disp('Weights');
  Mux : Mux  Inputs=15
      mask Display: e = 0.06;c1 = [120 150 230]/255;c2 = ([120 150 230]+0)/383;c3 = ([120 150 230]+128)/383;patch([0 1 1 0],[0 0 1 1],c1);patch([0 1 1 1-e 1-e 0+e],[0 0 1 1-e 0+e 0+e],c2);patch([0 0 1 1-e 0+e 0+e],[0 1 1 1-e 1-e 0+e],c3);plot([0 1 1 0 0],[0 0 1 1 0]);disp('Mux');
  dotprod{1..15} (15 alike) : neural/Weight Functions/dotprod
  "iz{1,1}" : Outport
      mask Display: e = 0.06;c1 = [120 230 180]/255;c2 = ([120 230 180]+0)/(256+128);c3 = ([120 230 180]+128)/(256+128);patch([0 1 1 0],[0 0 1 1],c1);patch([0 1 1 1-e 1-e 0+e],[0 0 1 1-e 0+e 0+e],c2);patch([0 0 1 1-e 0+e 0+e],[0 1 1 1-e 1-e 0+e],c3);plot([0 1 1 0 0],[0 0 1 1 0]);
  wires:
  "IW{1,1}(1,:)'"/1 -> dotprod1/1
  "pd{1,1}"/1 -> dotprod1/2, dotprod2/2, dotprod3/2, dotprod4/2, dotprod5/2, dotprod6/2, dotprod7/2, dotprod8/2, dotprod9/2, dotprod10/2, dotprod11/2, dotprod12/2, dotprod13/2, dotprod14/2, dotprod15/2
  dotprod1/1 -> Mux/1
  "IW{1,1}(2,:)'"/1 -> dotprod2/1
  dotprod2/1 -> Mux/2
  "IW{1,1}(3,:)'"/1 -> dotprod3/1
  dotprod3/1 -> Mux/3
  "IW{1,1}(4,:)'"/1 -> dotprod4/1
  dotprod4/1 -> Mux/4
  "IW{1,1}(5,:)'"/1 -> dotprod5/1
  dotprod5/1 -> Mux/5
  "IW{1,1}(6,:)'"/1 -> dotprod6/1
  dotprod6/1 -> Mux/6
  "IW{1,1}(7,:)'"/1 -> dotprod7/1
  dotprod7/1 -> Mux/7
  "IW{1,1}(8,:)'"/1 -> dotprod8/1
  dotprod8/1 -> Mux/8
  "IW{1,1}(9,:)'"/1 -> dotprod9/1
  dotprod9/1 -> Mux/9
  "IW{1,1}(10,:)'"/1 -> dotprod10/1
  dotprod10/1 -> Mux/10
  "IW{1,1}(11,:)'"/1 -> dotprod11/1
  dotprod11/1 -> Mux/11
  "IW{1,1}(12,:)'"/1 -> dotprod12/1
  dotprod12/1 -> Mux/12
  "IW{1,1}(13,:)'"/1 -> dotprod13/1
  dotprod13/1 -> Mux/13
  "IW{1,1}(14,:)'"/1 -> dotprod14/1
  dotprod14/1 -> Mux/14
  "IW{1,1}(15,:)'"/1 -> dotprod15/1
  dotprod15/1 -> Mux/15
  Mux/1 -> "iz{1,1}"/1

== system AFC_FFNN_trainscg_15_15_15_15_15_ctr_Nor_July_15/Feed-Forward Neural Network/Layer 2/Delays 1 ==
  "p{2}" : Inport  PortDimensions=15
      mask Display: e = 0.06;c1 = [120 230 180]/255;c2 = ([120 230 180]+0)/(256+128);c3 = ([120 230 180]+128)/(256+128);patch([0 1 1 0],[0 0 1 1],c1);patch([0 1 1 1-e 1-e 0+e],[0 0 1 1-e 0+e 0+e],c2);patch([0 0 1 1-e 0+e 0+e],[0 1 1 1-e 1-e 0+e],c3);plot([0 1 1 0 0],[0 0 1 1 0]);
  mux : Mux  Inputs=1
      mask Display: e = 0.06;c1 = [120 150 230]/255;c2 = ([120 150 230]+0)/383;c3 = ([120 150 230]+128)/383;patch([0 1 1 0],[0 0 1 1],c1);patch([0 1 1 1-e 1-e 0+e],[0 0 1 1-e 0+e 0+e],c2);patch([0 0 1 1-e 0+e 0+e],[0 1 1 1-e 1-e 0+e],c3);plot([0 1 1 0 0],[0 0 1 1 0]);disp('Mux')
  "pd{2,1}" : Outport
      mask Display: e = 0.06;c1 = [120 230 180]/255;c2 = ([120 230 180]+0)/(256+128);c3 = ([120 230 180]+128)/(256+128);patch([0 1 1 0],[0 0 1 1],c1);patch([0 1 1 1-e 1-e 0+e],[0 0 1 1-e 0+e 0+e],c2);patch([0 0 1 1-e 0+e 0+e],[0 1 1 1-e 1-e 0+e],c3);plot([0 1 1 0 0],[0 0 1 1 0]);
  wires:
  "p{2}"/1 -> mux/1
  mux/1 -> "pd{2,1}"/1
